simulink model "homeMobileManipulator"  (R2026a)
settings: Solver=ode4  StartTime=0  StopTime=Inf  FixedStep=cfg.rates.plant  MaxStep=cfg.rates.plant  AbsTol=1e-8
PostLoadFcn:
  | hmmSetup;
InitFcn:
  | hmmInitializeRun(bdroot);
values from neighbouring files (symbols this model uses):
  armJointLimits = zeros(numel(idx.arm), 2)    [hmmSetup.m]
  cfg = app.RunCfg    [HomeMobileManipulatorApp.m]    (also in HomeMobileManipulatorExample.m = params.cfg; hmmSetup.m = hmmConfig(); setupParams.m = data.cfg)
undefined symbols (not defined in the file or in its folder): actionQueueInit, actorNameTable, Angle, apertureMap, armPlanInit, Axis, basePlanInit, Custom, Extent, gray, gripperCoupling, invalidRayHits, movableRegistry, objectTargetInit, perceptionStatusInit, placeTargetInit, Position, robotStateInit, Sim3dSensor
libraries: robotmaniplib x20, robotcorelib x18, simulink x9, sim3dcameralib x6, sim3dgroundtruthsensorlib x4, dspmtrx3 x3, slpidlib x3, sim3dlib x3, hdlsllib x2, robotsim3dlib x1
(part 6 of 6)

== stateflow chart homeMobileManipulator/MobileManipulator/MobileBase/BaseSupervisor ==
  settings: updateMethod=DISCRETE  sampleTime=cfg.rates.supervisor
  state Operating
    state Idle
      en:
      Mode = M_IDLE;
      State = S_IDLE;
      FollowEnable = false;
      PlanRequest = false;
      ReplanRequest = false;
      Stalled = false;
      FollowTime = 0;
      PlanAttempts = uint8(0);
      FailureCode = F_OK;
    state AwaitPlan
      en:
      Mode = M_AWAIT;
      State = S_BUSY;
      FollowEnable = false;
      ReplanRequest = false;
      Stalled = false;
      planIdRef = BasePlan.RequestId;
      PlanAttempts = PlanAttempts + uint8(1);
      tWait = 0;
      PlanRequest = true;
      du:
      PlanRequest = false;
      tWait = tWait + dt;
      ex:
      PlanRequest = false;
    state Following
      en:
      Mode = M_FOLLOW;
      State = S_BUSY;
      FollowEnable = true;
      PlanRequest = false;
      ReplanRequest = false;
      Stalled = false;
      FollowTime = 0;
      tHold = 0;
      tProgress = 0;
      du:
      FollowTime = FollowTime + dt;
      vEq = sqrt(RobotState.BaseTwist(1)^2 + RobotState.BaseTwist(2)^2) ...
      + abs(RobotState.BaseTwist(3)) * rFoot;
      if vEq >= vStallMin
      tProgress = 0;
      else
      tProgress = tProgress + dt;
      end
      Stalled = tProgress >= tStall;
      if AtGoal
      tHold = tHold + dt;
      else
      tHold = 0;
      end
      ex:
      FollowEnable = false;
      settings: description=|
          | STALLED IS A SPEED TEST, which is what hmmDefineBuses line 384 has always published it
          | as: "Commanded to move but measured speed below cfg.track.stallSpeed."
          | 
          | It used to be a ratchet on DistanceToGoal instead - tProgress reset only when the
          | straight-line distance to the goal improved by
          | cfg.track.stallSpeed * cfg.track.stallTime = 0.02 * 2 = 0.04 m - and that condemns the
          | one manoeuvre every leg ends with. lateReverse arrives at a stand-off by pivoting as
          | stationary columns and then reversing in, and a terminal pivot NECESSARILY increases the
          | straight-line distance to the goal.
          | 
          | Measured over the 2.02 s before the run of 2026-10-04 was condemned: arc travelled
          | 0.3268 m, mean speed 0.162 m/s against a 0.020 threshold, mean yaw rate 0.521 rad/s, and
          | net closure 0.0196 m against the 0.04 m the ratchet demanded. The base was moving six
          | times faster than "stalled" while being called stalled. Because cfg.sup.retry.basePlan is
          | 2 and AwaitPlan increments PlanAttempts on entry, every leg tolerated exactly one such
          | stall, so the outcome was a coin flip. It lost that transfer: Stalled at 31.12 s ->
          | Recovering (FailureCode = F_PATH) -> PlanAttempts >= nPlanMax -> Holding (S_FAILED) at
          | 31.16 -> the task abandoned NavToPlace at 31.18 and cancelled the gripper, with the mug
          | still in the hand and the place pose perfectly reachable.
          | 
          | THE abs(wz)*rFoot TERM IS NOT OPTIONAL. The stationary pivot has vx = vy = 0 exactly, so
          | a plain hypot(vx,vy) test would call it stalled for the same reason the ratchet did. rFoot
          | is the footprint half-diagonal, hypot(halfLength, halfWidth) = 0.2485 m, so the pivot reads
          | 0.1295 m/s at the measured 0.521 rad/s, while a genuinely stuck base reads zero on all
          | three terms.
          | 
          | NOTHING IS LOST BY DROPPING THE DISTANCE TEST. A base driving at speed but never arriving
          | is still caught by FollowTime > tFollowMax on the transition out of this state, which is
          | the genuine stuck-base backstop; and AtGoal held for tGoalHold is what ends a successful
          | leg, on a transition with a lower execution order than the fault one.
          | 
          | DistanceToGoal (input port 5) IS DELIBERATELY RETAINED AND UNREAD. It is now the only
          | unused input on this chart. Deleting it renumbers CrossTrackError (6) and MinClearance (7),
          | and the chart inputs are wired by NUMBER inside MobileBase, so the deletion would silently
          | reconnect two live tracking-error guards to the wrong signals. An unused input costs
          | nothing; a silent miswiring of those guards costs a run that cannot be diagnosed.
    state Recovering
      en:
      Mode = M_RECOVER;
      State = S_BUSY;
      FollowEnable = false;
      PlanRequest = false;
      ReplanRequest = true;
      Stalled = false;
    state Holding
      en:
      Mode = M_HOLD;
      FollowEnable = false;
      PlanRequest = false;
      ReplanRequest = false;
      Stalled = false;
      FollowTime = 0;
    (default) -> Idle
    Idle -> Holding [order 2] : [BaseCommand.Valid && ...
        | BaseCommand.Request == REQ_HOLD]
        | {ServedRequestId = BaseCommand.RequestId;
        | State = S_IDLE;}
    Idle -> AwaitPlan [order 1] : [BaseCommand.Valid && ...
        | BaseCommand.Request == REQ_GOTO && ...
        | BaseCommand.RequestId ~= ServedRequestId]
        | {ServedRequestId = BaseCommand.RequestId;
        | PlanAttempts = uint8(0);
        | FailureCode = F_OK;}
    Operating -> Operating [order 1] : [BaseCommand.Cancel || BaseCommand.Stop]
        | {State = S_IDLE;}
    Holding -> AwaitPlan : [BaseCommand.Valid && ...
        | BaseCommand.Request == REQ_GOTO && ...
        | BaseCommand.RequestId ~= ServedRequestId]
        | {ServedRequestId = BaseCommand.RequestId;
        | PlanAttempts = uint8(0);
        | FailureCode = F_OK;}
    Recovering -> AwaitPlan [order 1] : [PlanAttempts < nPlanMax]
    AwaitPlan -> Following [order 1] : [BasePlan.RequestId ~= planIdRef && ...
        | BasePlan.Valid]
    AwaitPlan -> Recovering [order 2] : [BasePlan.RequestId ~= planIdRef && ...
        | ~BasePlan.Valid]
        | {FailureCode = BasePlan.FailureCode;}
    AwaitPlan -> Recovering [order 3] : [tWait > tPlanMax]{FailureCode = F_PATH;}
    Following -> Holding [order 1] : [tHold >= tGoalHold]
        | {State = S_DONE; FailureCode = F_OK;}
    Following -> Recovering [order 2] : [CrossTrackError > xTrackMax || Stalled || ...
        | FollowTime > tFollowMax]
        | {FailureCode = F_PATH;}
    Recovering -> Holding [order 2] : [PlanAttempts >= nPlanMax]
        | {State = S_FAILED;}
  state Stopped
    en:
    Mode = M_STOP;
    State = S_FAILED;
    FollowEnable = false;
    PlanRequest = false;
    ReplanRequest = false;
    Stalled = false;
    FollowTime = 0;
  (default) -> Operating
  Operating -> Stopped [order 1] : [SafetyStatus.EStop]
  data: BaseCommand input Bus: BaseCommand; SafetyStatus input Bus: SafetyStatus; BasePlan input Bus: BasePlan; AtGoal input boolean; CrossTrackError input double; Mode output uint8 =0; State output uint8 =0; ServedRequestId output uint32 =0; Stalled output boolean =0; ReplanRequest output boolean =0; PlanAttempts output uint8 =0; FailureCode output uint8 =0; PlanRequest output boolean =0; FollowEnable output boolean =0; FollowTime output double =0; planIdRef local uint32 =0; tWait local double =0; tHold local double =0; tProgress local double =0; dt constant double =cfg.rates.supervisor; REQ_GOTO constant uint8 =cfg.sup.baseReq.GOTO; REQ_HOLD constant uint8 =cfg.sup.baseReq.HOLD; M_IDLE constant uint8 =cfg.sup.base.IDLE; M_AWAIT constant uint8 =cfg.sup.base.AWAIT_PLAN; M_FOLLOW constant uint8 =cfg.sup.base.FOLLOWING; M_RECOVER constant uint8 =cfg.sup.base.RECOVERING; M_HOLD constant uint8 =cfg.sup.base.HOLDING; M_STOP constant uint8 =cfg.sup.base.STOPPED; S_IDLE constant uint8 =cfg.sup.st.IDLE; S_BUSY constant uint8 =cfg.sup.st.BUSY; S_DONE constant uint8 =cfg.sup.st.DONE; S_FAILED constant uint8 =cfg.sup.st.FAILED; F_OK constant uint8 =cfg.fail.OK; F_PATH constant uint8 =cfg.fail.PathPlanFailed; tPlanMax constant double =cfg.sup.timeout.basePlan; tFollowMax constant double =cfg.sup.timeout.follow; nPlanMax constant uint8 =cfg.sup.retry.basePlan; tStall constant double =cfg.track.stallTime; xTrackMax constant double =cfg.track.crossTrackMax; tGoalHold constant double =cfg.track.goalHoldTime; RobotState input Bus: RobotState; vStallMin constant double =cfg.track.stallSpeed; rFoot constant double =hypot(cfg.base.halfLength, cfg.base.halfWidth); vEq local double

== matlab function homeMobileManipulator/MobileManipulator/MobileBase/PathPlanning/BasePathSearch ==
  data: gridMatrix input; bplan output Bus: BasePlan; startPose input; goalPose input; carriedExtent input; requestId input; simTime input; planTemplate input; altGoalPose input
function bplan = BasePathSearch(gridMatrix, startPose, goalPose, carriedExtent, ...
                                requestId, simTime, planTemplate, altGoalPose)
%#codegen
% One SE(2) base path: inflate, search, score, time-parameterise.
%
% hmmPlanBasePath is extrinsic because every object it uses is a handle object
% with no block form - occupancyMap, stateSpaceSE2, validatorOccupancyMap,
% plannerBiRRT, navPath, pathmetrics - and because a sampling-based search takes
% a data-dependent number of iterations, which a fixed block diagram cannot
% express at all.
%
% planTemplate is what tells this block that bplan is a BasePlan bus. Its
% Waypoints and RefPose dimensions come from hmmDefineBuses, so a capacity change
% there propagates here without an edit.
coder.extrinsic('hmmPlanBasePath');

bplan = planTemplate;
% altGoalPose is the stand-off's partner heading; the planner plans both and keeps the cheaper
% drive, and bplan.GoalPose records which - PathFollowing judges arrival against that.
bplan = hmmPlanBasePath(gridMatrix, startPose, goalPose, carriedExtent, ...
    requestId, simTime, planTemplate, altGoalPose);
end

== stateflow chart homeMobileManipulator/MobileManipulator/Manipulator/ArmSupervisor ==
  settings: updateMethod=DISCRETE  sampleTime=cfg.rates.supervisor
  state Operating
    state Idle
      en:
      Mode = M_IDLE;
      State = S_IDLE;
      PlanRequest = false;
      TaskSpaceMode = false;
      StowSelect = true;
      HoldSelect = false;
      MoveTime = 0;
      ApproachOffset = 0;
      ArmMode = MODE_PICK;
      PlanAttempts = uint8(0);
      FailureCode = F_OK;
    state AwaitPlan
      en:
      Mode = M_AWAIT;
      State = S_BUSY;
      TaskSpaceMode = false;
      % HOLD WHERE THE ARM IS, DO NOT COMMAND STOW. This state used to set StowSelect
      % true, which ReferenceSelect resolves to a hard cfg.arm.stowConfig command. On the
      % FIRST plan request that is a no-op because the arm is already stowed, but on every
      % later request - the refinement replan, and the place replan after a retreat - the arm
      % is somewhere else, so it was commanded 3.16 rad away for the one tick spent here.
      % JointSpaceTrack is a dynamic block carrying its own integrated state, so 20 ms of that
      % step left it accelerating toward stow and the tool strayed 63.6 mm off a 41.6 mm move
      % before coming back. HoldSelect commands the MEASURED ArmJointPos instead, which is a
      % null step by construction. Holding deliberately does NOT clear it, the same way it does
      % not clear StowSelect: if a plan never arrives the arm should stay put, not lurch.
      StowSelect = false;
      HoldSelect = true;
      MoveTime = 0;
      ApproachOffset = 0;
      if ArmCommand.Request == REQ_PLAN_PLACE
      ArmMode = MODE_PLACE;
      elseif ArmCommand.Request == REQ_STOW
      % A STOW IS PLANNED NOW (hmmScreenArmPlan, ARM_MODE_STOW) - see the AwaitPlan -> Stowing fallback.
      ArmMode = MODE_STOW;
      else
      ArmMode = MODE_PICK;
      end
      planIdRef = ArmPlan.RequestId;
      PlanAttempts = PlanAttempts + uint8(1);
      tWait = 0;
      PlanRequest = true;
      du:
      PlanRequest = false;
      tWait = tWait + dt;
      ex:
      PlanRequest = false;
    state MovingFree
      en:
      Mode = M_MOVING;
      State = S_BUSY;
      PlanRequest = false;
      TaskSpaceMode = false;
      StowSelect = false;
      HoldSelect = false;
      % THE FREE MOVE ENDS AT THE STANDOFF, so that is where the offset stands
      % when this phase finishes. hmmScreenArmPlan plans stow -> pre-grasp rather than
      % stow -> grasp, and ApproachConstrained ramps the offset DOWN from whatever it
      % inherits: inheriting 0 would satisfy its own exit guard on the first tick, so
      % the approach would report S_DONE without moving and leave the tool the whole
      % standoff short of the grasp. The value is unused while this state is active because
      % TaskSpaceMode is false; it is set here because this is where it becomes true.
      %
      % IT COMES FROM THE PLAN, NOT FROM depthDefault, BECAUSE THE PICK'S STANDOFF IS SEARCHED.
      % hmmScreenArmPlan walks cfg.sup.approachDepthLadder down from cfg.sup.approachDepthPickMax
      % and reports the rung it actually solved PregraspConfig at as ArmPlan.ApproachDepth, so
      % the constant is correct only for a place. Reading the constant here while the planner had
      % parked the tool 0.240 m up would leave ApproachConstrained ramping 0.080 of a 0.240 gap
      % and closing the jaws 0.160 m above the object - and it would look HEALTHY, because the
      % ramp reaches its own target and the exit guard above is met on time.
      %
      % NOT A PREFERENCE BETWEEN TWO SOURCES. ArmPlan.ApproachDepth is the standoff the pregrasp
      % pose was SOLVED at, so it is a fact about where the arm physically is, not a request that
      % something else may override. The guard is belt and braces: the only entry into this state
      % already requires ArmPlan.Valid, but a state action should not depend silently on that.
      if ArmPlan.Valid && ArmPlan.ApproachDepth > 0
      ApproachOffset = ArmPlan.ApproachDepth;
      else
      ApproachOffset = depthDefault;
      end
      MoveTime = 0;
      tPhase = 0;
      du:
      MoveTime = MoveTime + dt;
      tPhase = tPhase + dt;
    state Stowing
      en:
      Mode = M_STOWING;
      State = S_BUSY;
      PlanRequest = false;
      TaskSpaceMode = false;
      StowSelect = true;
      HoldSelect = false;
      MoveTime = 0;
      ApproachOffset = 0;
      tPhase = 0;
      du:
      tPhase = tPhase + dt;
    state ApproachConstrained
      en:
      Mode = M_APPROACH;
      State = S_BUSY;
      PlanRequest = false;
      TaskSpaceMode = true;
      StowSelect = false;
      HoldSelect = false;
      tPhase = 0;
      depthTarget = 0;
      du:
      tPhase = tPhase + dt;
      if ApproachOffset > depthTarget + approachRate * dt
      ApproachOffset = ApproachOffset - approachRate * dt;
      else
      ApproachOffset = depthTarget;
      end
    state Retreating
      en:
      Mode = M_RETREAT;
      State = S_BUSY;
      PlanRequest = false;
      TaskSpaceMode = true;
      StowSelect = false;
      HoldSelect = false;
      tPhase = 0;
      if ArmCommand.ApproachDepth > 0
      depthTarget = ArmCommand.ApproachDepth;
      else
      depthTarget = depthDefault;
      end
      du:
      tPhase = tPhase + dt;
      if ApproachOffset < depthTarget - approachRate * dt
      ApproachOffset = ApproachOffset + approachRate * dt;
      else
      ApproachOffset = depthTarget;
      end
    state Holding
      en:
      Mode = M_HOLD;
      PlanRequest = false;
    (default) -> Idle
    Idle -> (junction 57) : [ArmCommand.Valid && ...
        | ArmCommand.RequestId ~= ServedRequestId]
        | {ServedRequestId = ArmCommand.RequestId;
        | PlanAttempts = uint8(0);
        | FailureCode = F_OK;}
    (junction 57) -> Retreating [order 3] : [ArmCommand.Request == REQ_RETREAT]
    (junction 57) -> Stowing [order 4] : [ArmCommand.Request == REQ_STOW]
    (junction 57) -> ApproachConstrained [order 2] : [ArmCommand.Request == REQ_APPROACH]
    (junction 57) -> Holding [order 5] : [ArmCommand.Request == REQ_HOLD]
        | {State = S_IDLE;}
    (junction 57) -> Holding [order 6] : {State = S_FAILED; FailureCode = F_UNKNOWN;}
    Holding -> (junction 57) [order 1] : [ArmCommand.Valid && ...
        | ArmCommand.RequestId ~= ServedRequestId]
        | {ServedRequestId = ArmCommand.RequestId;
        | PlanAttempts = uint8(0);
        | FailureCode = F_OK;}
    (junction 57) -> AwaitPlan [order 1] : [ArmCommand.Request == REQ_PLAN_PICK || ...
        | ArmCommand.Request == REQ_PLAN_PLACE || ...
        | ArmCommand.Request == REQ_STOW]
    Operating -> Operating [order 1] : [ArmCommand.Cancel || ArmCommand.Stop]
        | {State = S_IDLE;}
    Holding -> AwaitPlan [order 2] : [State == S_BUSY]
    AwaitPlan -> MovingFree [order 1] : [ArmPlan.RequestId ~= planIdRef && ...
        | ArmPlan.Valid]
    AwaitPlan -> Stowing [order 3] : [ArmMode == MODE_STOW && tWait > tPlanMax]
      settings: description=STOW FALLBACK on a plan timeout, as above.
    AwaitPlan -> Stowing [order 2] : [ArmMode == MODE_STOW && ...
        | ArmPlan.RequestId ~= planIdRef && ...
        | ~ArmPlan.Valid && ...
        | PlanAttempts >= 2 * nPlanMax]
      settings: description=STOW FALLBACK: no planned stow, so the direct joint-space stow it replaced. Never worse than before; logged as the plan failure code.
    AwaitPlan -> Holding [order 7] : [tWait > tPlanMax]
        | {FailureCode = F_ARM; State = S_FAILED;}
    AwaitPlan -> Holding [order 4] : [ArmPlan.RequestId ~= planIdRef && ...
        | ~ArmPlan.Valid && ...
        | (PlanAttempts < nPlanMax || (ArmMode == MODE_STOW && PlanAttempts < 2 * nPlanMax))]
        | {FailureCode = ArmPlan.FailureCode;}
    AwaitPlan -> Holding [order 5] : [ArmPlan.RequestId ~= planIdRef && ...
        | ~ArmPlan.Valid]
        | {FailureCode = ArmPlan.FailureCode;
        | State = S_FAILED;}
    AwaitPlan -> Holding [order 6] : [tWait > tPlanMax && ...
        | PlanAttempts < nPlanMax]
        | {FailureCode = F_ARM;}
    Stowing -> Holding [order 2] : [tPhase > tStowMax]
        | {State = S_FAILED; FailureCode = F_ARM;}
    Stowing -> Holding [order 1] : [Settled && tPhase >= tSettleMin]
        | {State = S_DONE; FailureCode = F_OK;}
    ApproachConstrained -> Holding [order 1] : [ApproachOffset <= depthTarget && Settled && ...
        | tPhase >= tSettleMin]
        | {State = S_DONE; FailureCode = F_OK;}
    ApproachConstrained -> Holding [order 2] : [tPhase > tApproachMax]
        | {State = S_FAILED; FailureCode = F_ARM;}
    ApproachConstrained -> Holding [order 3] : [TrackingError > xTrackMax]
        | {State = S_FAILED; FailureCode = F_ARM;}
    Retreating -> Holding [order 1] : [ApproachOffset >= depthTarget && Settled && ...
        | tPhase >= tSettleMin]
        | {State = S_DONE; FailureCode = F_OK;}
    Retreating -> Holding [order 2] : [tPhase > tApproachMax]
        | {State = S_FAILED; FailureCode = F_ARM;}
    Retreating -> Holding [order 3] : [TrackingError > xTrackMax]
        | {State = S_FAILED; FailureCode = F_ARM;}
    MovingFree -> Holding [order 3] : [TrackingError > xTrackMax]
        | {State = S_FAILED; FailureCode = F_ARM;}
    MovingFree -> Holding [order 1] : [MoveTime >= ArmPlan.Duration && Settled && ...
        | tPhase >= tSettleMin]
        | {State = S_DONE; FailureCode = F_OK;}
    MovingFree -> Holding [order 2] : [tPhase > tMoveMax]
        | {State = S_FAILED; FailureCode = F_ARM;}
  state Stopped
    en:
    Mode = M_STOP;
    State = S_FAILED;
    PlanRequest = false;
  (default) -> Operating
  Operating -> Stopped [order 1] : [SafetyStatus.EStop]
  data: ArmCommand input Bus: ArmCommand; SafetyStatus input Bus: SafetyStatus; ArmPlan input Bus: ArmPlan; Settled input boolean; TrackingError input double; PlanRequest output boolean =0; ArmMode output uint8 =0; MoveTime output double =0; TaskSpaceMode output boolean =0; ApproachOffset output double =0; StowSelect output boolean =0; Mode output uint8 =0; State output uint8 =0; ServedRequestId output uint32 =0; PlanAttempts output uint8 =0; FailureCode output uint8 =0; planIdRef local uint32 =0; tWait local double =0; tPhase local double =0; depthTarget local double =0; dt constant double =cfg.rates.supervisor; REQ_PLAN_PICK constant uint8 =cfg.sup.armReq.PLAN_PICK; REQ_PLAN_PLACE constant uint8 =cfg.sup.armReq.PLAN_PLACE; REQ_APPROACH constant uint8 =cfg.sup.armReq.APPROACH; REQ_RETREAT constant uint8 =cfg.sup.armReq.RETREAT; REQ_STOW constant uint8 =cfg.sup.armReq.STOW; REQ_HOLD constant uint8 =cfg.sup.armReq.HOLD; M_IDLE constant uint8 =cfg.sup.arm.IDLE; M_AWAIT constant uint8 =cfg.sup.arm.AWAIT_PLAN; M_MOVING constant uint8 =cfg.sup.arm.MOVING_FREE; M_APPROACH constant uint8 =cfg.sup.arm.APPROACH; M_RETREAT constant uint8 =cfg.sup.arm.RETREATING; M_STOWING constant uint8 =cfg.sup.arm.STOWING; M_HOLD constant uint8 =cfg.sup.arm.HOLDING; M_STOP constant uint8 =cfg.sup.arm.STOPPED; S_IDLE constant uint8 =cfg.sup.st.IDLE; S_BUSY constant uint8 =cfg.sup.st.BUSY; S_DONE constant uint8 =cfg.sup.st.DONE; S_FAILED constant uint8 =cfg.sup.st.FAILED; F_OK constant uint8 =cfg.fail.OK; F_ARM constant uint8 =cfg.fail.ArmPlanFailed; F_UNKNOWN constant uint8 =cfg.fail.UnknownAction; MODE_PICK constant uint8 =cfg.plan.ARM_MODE_PICK; MODE_PLACE constant uint8 =cfg.plan.ARM_MODE_PLACE; tPlanMax constant double =cfg.sup.timeout.armPlan; tMoveMax constant double =cfg.sup.timeout.armMove; tApproachMax constant double =cfg.sup.timeout.approach; tStowMax constant double =cfg.sup.timeout.stow; nPlanMax constant uint8 =cfg.sup.retry.armPlan; xTrackMax constant double =cfg.safety.trackErrMax; depthDefault constant double =cfg.sup.approachDepth; approachRate constant double =cfg.sup.approachRate; tSettleMin constant double =3 * cfg.rates.supervisor; HoldSelect output boolean; MODE_STOW constant uint8 =cfg.plan.ARM_MODE_STOW

== matlab function homeMobileManipulator/MobileManipulator/Manipulator/MotionPlanning/ScreenAndPlan ==
  data: objectTarget input; aplan output Bus: ArmPlan; placeTarget input; mode input; robotConfig input; tfArmFromMap input; graspConfigs input; poseErrors input; manipulability input; graspPoses input; requestId input; simTime input; planTemplate input
function aplan = ScreenAndPlan(objectTarget, placeTarget, mode, robotConfig, ...
                               tfArmFromMap, graspConfigs, poseErrors, manipulability, ...
                               graspPoses, requestId, simTime, planTemplate)
%#codegen
% THE KINEMATICS ARE BLOCKS, NOT CODE. The three Candidate_k subsystems each hold
% an Inverse Kinematics block, a Get Jacobian block and a Reciprocal Condition
% block, and MapToArmFrame is a Get Transform block, so this function is handed a
% solved configuration, a residual and a manipulability index per candidate. What
% is left - screening, collision rejection, manipulatorRRT and contopptraj - has
% no block form in any installed library.
%
% planTemplate IS THE PREVIOUS ANSWER, fed back through PrevPlan. It carries the
% element types so nothing here decides them, and it carries the RequestId that
% lets hmmScreenArmPlan return the held plan instead of paying for the same
% search on every tick of a held enable.
%
% THE OUTPUT IS TYPED BEFORE THE EXTRINSIC CALL. An extrinsic function returns
% mxArray, so aplan must already be a fully typed ArmPlan value or the block
% cannot infer its output bus.
coder.extrinsic('hmmScreenArmPlan');

aplan = planTemplate;

aplan = hmmScreenArmPlan(objectTarget, placeTarget, mode, robotConfig, ...
                         tfArmFromMap, graspConfigs, poseErrors, manipulability, ...
                         graspPoses, requestId, simTime, planTemplate);
end

== stateflow chart homeMobileManipulator/MobileManipulator/Gripper/GripperSupervisor ==
  settings: updateMethod=DISCRETE  sampleTime=cfg.rates.supervisor
  state Operating
    state Open
      en:
      Mode = M_OPEN;
      GraspRequestCmd = false;
      CloseRequested = false;
      Grasped = false;
    state Closing
      en:
      Mode = M_CLOSING;
      State = S_BUSY;
      GraspRequestCmd = false;
      CloseRequested = true;
      tPhase = 0;
      tStall = 0;
      aperturePrev = Aperture;
      ApertureCmd = Aperture;
      if GripperCommand.TargetAperture > 0
      aTarget = GripperCommand.TargetAperture;
      else
      aTarget = aClosed;
      end
      du:
      tPhase = tPhase + dt;
      if ApertureCmd > aTarget + aRate * dt
      ApertureCmd = ApertureCmd - aRate * dt;
      else
      ApertureCmd = aTarget;
      end
      if tPhase > tSettle && abs(Aperture - aperturePrev) < aStallEps
      tStall = tStall + dt;
      else
      tStall = 0;
      end
      aperturePrev = Aperture;
    state Closed
      en:
      Mode = M_CLOSED;
      State = S_BUSY;
      GraspRequestCmd = true;
      CloseRequested = true;
      tPhase = 0;
      du:
      tPhase = tPhase + dt;
    state GraspValidated
      en:
      Mode = M_VALIDATED;
      State = S_DONE;
      GraspRequestCmd = true;
      CloseRequested = true;
      Grasped = true;
      Slipped = false;
      FailureCode = F_OK;
      tPhase = 0;
      du:
      tPhase = tPhase + dt;
    state Opening
      en:
      Mode = M_OPENING;
      State = S_BUSY;
      GraspRequestCmd = false;
      CloseRequested = false;
      Grasped = false;
      tPhase = 0;
      ApertureCmd = Aperture;
      if GripperCommand.TargetAperture > 0
      aTarget = GripperCommand.TargetAperture;
      else
      aTarget = aOpen;
      end
      du:
      tPhase = tPhase + dt;
      if ApertureCmd < aTarget - aRate * dt
      ApertureCmd = ApertureCmd + aRate * dt;
      else
      ApertureCmd = aTarget;
      end
    (default) -> Open
    Open -> Opening [order 2] : [GripperCommand.Valid && ...
        | GripperCommand.Request == REQ_OPEN && ...
        | GripperCommand.RequestId ~= ServedRequestId]
        | {ServedRequestId = GripperCommand.RequestId;
        | FailureCode = F_OK;}
    Opening -> Open [order 1] : [ApertureCmd >= aTarget - aTol && ...
        | tPhase >= tSettle]
        | {State = S_DONE;}
    Open -> Closing [order 1] : [GripperCommand.Valid && ...
        | GripperCommand.Request == REQ_CLOSE && ...
        | GripperCommand.RequestId ~= ServedRequestId]
        | {ServedRequestId = GripperCommand.RequestId;
        | FailureCode = F_OK;}
    Closing -> Closed [order 1] : [tStall >= tSettle || ...
        | (ApertureCmd <= aTarget + aTol && tPhase >= tSettle)]
    Closed -> Opening [order 1] : [GripperCommand.Valid && ...
        | GripperCommand.Request == REQ_OPEN && ...
        | GripperCommand.RequestId ~= ServedRequestId]
        | {ServedRequestId = GripperCommand.RequestId;
        | FailureCode = F_OK;}
    Closed -> GraspValidated [order 2] : [IsGrasped && ...
        | AttachedActorId ~= noneActor && ...
        | tPhase >= tSettle]
    GraspValidated -> Opening [order 2] : [GripperCommand.Valid && ...
        | GripperCommand.Request == REQ_OPEN && ...
        | GripperCommand.RequestId ~= ServedRequestId]
        | {ServedRequestId = GripperCommand.RequestId;
        | FailureCode = F_OK;}
  state Faulted
    en:
    Mode = M_FAULTED;
    CloseRequested = false;
  (default) -> Operating
  Open -> Faulted [order 3] : [GripperCommand.Valid && ...
      | GripperCommand.RequestId ~= ServedRequestId]
      | {ServedRequestId = GripperCommand.RequestId;
      | State = S_FAILED; FailureCode = F_UNKNOWN;}
  Closing -> Faulted [order 2] : [tPhase > tGripMax]
      | {State = S_FAILED;
      | FailureCode = F_NOTGRASP;}
  Operating -> Faulted [order 2] : [(GripperCommand.Cancel || GripperCommand.Stop) && ...
      | ~in(Operating.GraspValidated)]
      | {State = S_IDLE;}
  Operating -> Faulted [order 1] : [SafetyStatus.EStop]{State = S_FAILED;}
  Closed -> Faulted [order 3] : [tPhase > tGripMax]
      | {State = S_FAILED;
      | FailureCode = F_NOTGRASP;}
  GraspValidated -> Faulted [order 1] : [~IsGrasped]
      | {State = S_FAILED; FailureCode = F_NOTGRASP;
      | Slipped = true; Grasped = false;}
  Opening -> Faulted [order 2] : [tPhase > tGripMax]
      | {State = S_FAILED;
      | FailureCode = F_NOTGRASP;}
  Faulted -> Opening : [~SafetyStatus.EStop && ...
      | ~GripperCommand.Stop && ...
      | GripperCommand.Valid && ...
      | GripperCommand.Request == REQ_OPEN && ...
      | GripperCommand.RequestId ~= ServedRequestId]
      | {ServedRequestId = GripperCommand.RequestId;
      | FailureCode = F_OK; Slipped = false;}
  data: GripperCommand input Bus: GripperCommand; SafetyStatus input Bus: SafetyStatus; Aperture input double; IsGrasped input boolean; AttachedActorId input uint8; ApertureCmd output double =cfg.gripper.maxOpenPos; GraspRequestCmd output boolean =0; CloseRequested output boolean =0; Mode output uint8 =cfg.sup.grip.OPEN; State output uint8 =cfg.sup.st.IDLE; ServedRequestId output uint32 =0; Grasped output boolean =0; Slipped output boolean =0; FailureCode output uint8 =0; tPhase local double =0; tStall local double =0; aperturePrev local double =0; aTarget local double =0; dt constant double =cfg.rates.supervisor; REQ_OPEN constant uint8 =cfg.sup.gripReq.OPEN; REQ_CLOSE constant uint8 =cfg.sup.gripReq.CLOSE; M_OPEN constant uint8 =cfg.sup.grip.OPEN; M_CLOSING constant uint8 =cfg.sup.grip.CLOSING; M_CLOSED constant uint8 =cfg.sup.grip.CLOSED; M_VALIDATED constant uint8 =cfg.sup.grip.VALIDATED; M_OPENING constant uint8 =cfg.sup.grip.OPENING; M_FAULTED constant uint8 =cfg.sup.grip.FAULTED; S_IDLE constant uint8 =cfg.sup.st.IDLE; S_BUSY constant uint8 =cfg.sup.st.BUSY; S_DONE constant uint8 =cfg.sup.st.DONE; S_FAILED constant uint8 =cfg.sup.st.FAILED; F_OK constant uint8 =cfg.fail.OK; F_NOTGRASP constant uint8 =cfg.fail.NotGraspable; F_UNKNOWN constant uint8 =cfg.fail.UnknownAction; aRate constant double =cfg.gripper.apertureRateMax; aTol constant double =cfg.gripper.apertureTol; aOpen constant double =cfg.gripper.maxOpenPos; aClosed constant double =cfg.gripper.minOpenPos; aStallEps constant double =0.1 * cfg.gripper.apertureRateMax * cfg.rates.supervisor; tGripMax constant double =cfg.sup.timeout.grip; tSettle constant double =cfg.sup.graspSettle; noneActor constant uint8 =cfg.actor.noneId

== matlab function homeMobileManipulator/MobileManipulator/Plant/ChaseCamera/ChaseBoom ==
  data: Tchassis input; T output
function T = ChaseBoom(Tchassis)
%CHASEBOOM The chase camera's pose, behind and above the chassis on a boom that shortens
%   in front of a wall - see hmmChaseBoom. Display only.
coder.extrinsic('hmmChaseBoom');
T = zeros(4, 4);
T = hmmChaseBoom(Tchassis);

== matlab function homeMobileManipulator/MobileManipulator/Plant/RobotActor/ReleaseSettle ==
  data: IsGrasped input; SettleDz output; TargetActorId input; RobotConfig input
function SettleDz = ReleaseSettle(IsGrasped, TargetActorId, RobotConfig)
%RELEASESETTLE Fake gravity at release: rest the prop just let go on the surface beneath it.
%   The plant has no physics - Sim3D's detach asks for gravity on the released prop, but the
%   multi-part prop meshes have Static children, so the engine never lets them fall. On the
%   falling edge of IsGrasped (the step the Simulation 3D Robot block detaches) the prop that
%   was held is handed to hmmSettleProp with this step's RobotConfig - the actor's own
%   Translation is still end-effector-relative on the detach step, so the prop's world position
%   is computed from FK and the frozen attach offset - and rested on the swept shell surface under its
%   footprint and prints the correction. PLANT-SIDE ONLY: SettleDz feeds nothing in control.
coder.extrinsic('hmmSettleProp');
persistent wasGrasped heldId
if isempty(wasGrasped)
    wasGrasped = false;
    heldId = 0;
end
SettleDz = 0;
if IsGrasped
    heldId = double(TargetActorId);
elseif wasGrasped && heldId > 0
    SettleDz = hmmSettleProp(heldId, double(RobotConfig(:))');
    heldId = 0;
end
wasGrasped = logical(IsGrasped);
